simulink model "q1s"  (R2022a)
settings: Solver=VariableStepAuto  StartTime=0.0  StopTime=10.0  RelTol=1e-3
settings Model: Creator=giova  LastModifiedBy=giova

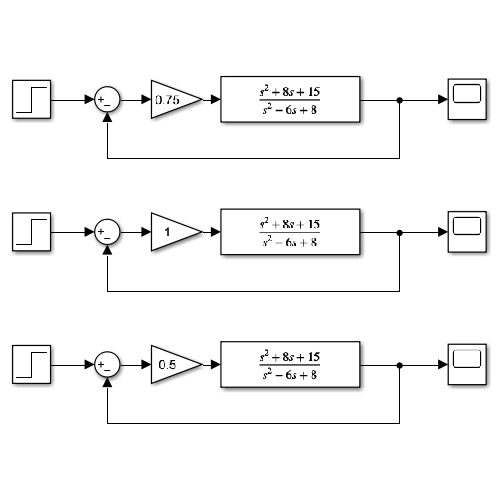
[thumbnail: Simulink's stored preview of the top-level diagram]
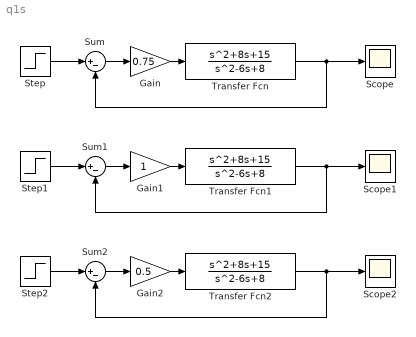
== system q1s ==
  Gain : Gain  Gain=0.75
  Gain1 : Gain
  Gain2 : Gain  Gain=0.5
  Scope : Scope
  Scope1 : Scope
  Scope2 : Scope
  Step : Step  After=5  SampleTime=0
  Step1 : Step  After=5  SampleTime=0
  Step2 : Step  After=5  SampleTime=0
  Sum : Sum  Inputs=|+-
  Sum1 : Sum  Inputs=|+-
  Sum2 : Sum  Inputs=|+-
  Transfer Fcn : TransferFcn  Numerator=[1 8 15]  Denominator=[1 -6 8]
  Transfer Fcn1 : TransferFcn  Numerator=[1 8 15]  Denominator=[1 -6 8]
  Transfer Fcn2 : TransferFcn  Numerator=[1 8 15]  Denominator=[1 -6 8]
  wires:
  Transfer Fcn/1 -> Sum/2, Scope/1
  Step/1 -> Sum/1
  Sum/1 -> Gain/1
  Gain/1 -> Transfer Fcn/1
  Sum1/1 -> Gain1/1
  Gain1/1 -> Transfer Fcn1/1
  Transfer Fcn1/1 -> Sum1/2, Scope1/1
  Step1/1 -> Sum1/1
  Sum2/1 -> Gain2/1
  Gain2/1 -> Transfer Fcn2/1
  Transfer Fcn2/1 -> Sum2/2, Scope2/1
  Step2/1 -> Sum2/1
